simulink model "StampFly_StudentBlocks"  (R2026b)
settings: Solver=VariableStepAuto
undefined symbols (not defined in the file): Bottom, Official
(part 4 of 6)

== system StampFly_StudentBlocks/FlightSequence/OfficialTakeoffHover400/TakeoffHoverControl400/PitchRatePID ==
  Error : Inport
  Dt : Inport  Port=2
  Enable : Inport  Port=3
  Reset : Inport  Port=4
  PreviousError : Inport  Port=5
  ApplyKp : Product
  DMemory : UnitDelay  InitialCondition=single(0)  SampleTime=Official.Step
  DerivativeDenominator : Sum
  DerivativeErrorProduct : Product
  DerivativeErrorTerm : Product  Inputs=*/
  DerivativePreviousNumerator : Sum  Inputs=+-
  DerivativeUpdate : Sum
  DivideTi : Product  Inputs=*/
  EMemory : UnitDelay  InitialCondition=single(0)  SampleTime=Official.Step
  ErrorDifference : Sum  Inputs=+-
  ErrorPair : Sum
  ErrorPairDt : Product
  Eta : Constant  Value=single(0.125)
  EtaTd : Product
  HalfIntegral : Gain  Gain=single(.5)
  IMemory : UnitDelay  InitialCondition=single(0)  SampleTime=Official.Step
  IntegralLimit : Saturate  UpperLimit=single(30000)  LowerLimit=single(-30000)
  IntegralUpdate : Sum
  Kp : Constant  Value=single(0.949999988)
  PIDTerms : Sum  Inputs=+++
  PreviousDerivativeProduct : Product
  PreviousDerivativeTerm : Product  Inputs=*/
  Select_dnext : Switch  Criteria=u2 ~= 0  SaturateOnIntegerOverflow=off  InputSameDT=off
  Select_dp : Switch  Criteria=u2 ~= 0  SaturateOnIntegerOverflow=off  InputSameDT=off
  Select_enext : Switch  Criteria=u2 ~= 0  SaturateOnIntegerOverflow=off  InputSameDT=off
  Select_ep : Switch  Criteria=u2 ~= 0  SaturateOnIntegerOverflow=off  InputSameDT=off
  Select_inext : Switch  Criteria=u2 ~= 0  SaturateOnIntegerOverflow=off  InputSameDT=off
  Select_ip : Switch  Criteria=u2 ~= 0  SaturateOnIntegerOverflow=off  InputSameDT=off
  Select_output : Switch  Criteria=u2 ~= 0  SaturateOnIntegerOverflow=off  InputSameDT=off
  Select_ynext : Switch  Criteria=u2 ~= 0  SaturateOnIntegerOverflow=off  InputSameDT=off
  Td : Constant  Value=single(0.0250000004)
  Ti : Constant  Value=single(0.699999988)
  TwiceEtaTd : Gain  Gain=single(2)
  TwiceTd : Gain  Gain=single(2)
  YMemory : UnitDelay  InitialCondition=single(0)  SampleTime=Official.Step
  Zero : Constant  Value=single(0)
  Output : Outport
  wires:
  Enable/1 -> Select_output/2, Select_inext/2, Select_dnext/2, Select_enext/2, Select_ynext/2
  ApplyKp/1 -> Select_ynext/1, Select_output/1
  YMemory/1 -> Select_ynext/3, Select_output/3
  Select_ynext/1 -> YMemory/1
  Select_output/1 -> Output/1
  Select_enext/1 -> EMemory/1
  Select_dnext/1 -> DMemory/1
  Select_inext/1 -> IMemory/1
  PIDTerms/1 -> ApplyKp/2
  Kp/1 -> ApplyKp/1
  DerivativeUpdate/1 -> PIDTerms/3, Select_dnext/1
  IntegralLimit/1 -> PIDTerms/2, Select_inext/1
  DerivativeErrorTerm/1 -> DerivativeUpdate/2
  PreviousDerivativeTerm/1 -> DerivativeUpdate/1
  DerivativeErrorProduct/1 -> DerivativeErrorTerm/1
  ErrorDifference/1 -> DerivativeErrorProduct/2
  TwiceTd/1 -> DerivativeErrorProduct/1
  DerivativeDenominator/1 -> PreviousDerivativeTerm/2, DerivativeErrorTerm/2
  PreviousDerivativeProduct/1 -> PreviousDerivativeTerm/1
  Select_dp/1 -> PreviousDerivativeProduct/2, Select_dnext/3
  DerivativePreviousNumerator/1 -> PreviousDerivativeProduct/1
  TwiceEtaTd/1 -> DerivativePreviousNumerator/1, DerivativeDenominator/1
  EtaTd/1 -> TwiceEtaTd/1
  Td/1 -> EtaTd/2, TwiceTd/1
  Eta/1 -> EtaTd/1
  IntegralUpdate/1 -> IntegralLimit/1
  DivideTi/1 -> IntegralUpdate/2
  Select_ip/1 -> Select_inext/3, IntegralUpdate/1
  Ti/1 -> DivideTi/2
  HalfIntegral/1 -> DivideTi/1
  ErrorPairDt/1 -> HalfIntegral/1
  ErrorPair/1 -> ErrorPairDt/2
  Dt/1 -> ErrorPairDt/1, DerivativeDenominator/2, DerivativePreviousNumerator/2
  Select_ep/1 -> Select_enext/3, ErrorPair/2, ErrorDifference/2
  Error/1 -> ErrorPair/1, ErrorDifference/1, PIDTerms/1, Select_enext/1
  EMemory/1 -> Select_ep/3
  PreviousError/1 -> Select_ep/1
  DMemory/1 -> Select_dp/3
  IMemory/1 -> Select_ip/3
  Reset/1 -> Select_ip/2, Select_dp/2, Select_ep/2
  Zero/1 -> Select_ip/1, Select_dp/1

== system StampFly_StudentBlocks/FlightSequence/OfficialTakeoffHover400/TakeoffHoverControl400/RollAnglePID ==
  Error : Inport
  Dt : Inport  Port=2
  Enable : Inport  Port=3
  Reset : Inport  Port=4
  PreviousError : Inport  Port=5
  ApplyKp : Product
  DMemory : UnitDelay  InitialCondition=single(0)  SampleTime=Official.Step
  DerivativeDenominator : Sum
  DerivativeErrorProduct : Product
  DerivativeErrorTerm : Product  Inputs=*/
  DerivativePreviousNumerator : Sum  Inputs=+-
  DerivativeUpdate : Sum
  DivideTi : Product  Inputs=*/
  EMemory : UnitDelay  InitialCondition=single(0)  SampleTime=Official.Step
  ErrorDifference : Sum  Inputs=+-
  ErrorPair : Sum
  ErrorPairDt : Product
  Eta : Constant  Value=single(0.125)
  EtaTd : Product
  HalfIntegral : Gain  Gain=single(.5)
  IMemory : UnitDelay  InitialCondition=single(0)  SampleTime=Official.Step
  IntegralLimit : Saturate  UpperLimit=single(30000)  LowerLimit=single(-30000)
  IntegralUpdate : Sum
  Kp : Constant  Value=single(5)
  PIDTerms : Sum  Inputs=+++
  PreviousDerivativeProduct : Product
  PreviousDerivativeTerm : Product  Inputs=*/
  Select_dnext : Switch  Criteria=u2 ~= 0  SaturateOnIntegerOverflow=off  InputSameDT=off
  Select_dp : Switch  Criteria=u2 ~= 0  SaturateOnIntegerOverflow=off  InputSameDT=off
  Select_enext : Switch  Criteria=u2 ~= 0  SaturateOnIntegerOverflow=off  InputSameDT=off
  Select_ep : Switch  Criteria=u2 ~= 0  SaturateOnIntegerOverflow=off  InputSameDT=off
  Select_inext : Switch  Criteria=u2 ~= 0  SaturateOnIntegerOverflow=off  InputSameDT=off
  Select_ip : Switch  Criteria=u2 ~= 0  SaturateOnIntegerOverflow=off  InputSameDT=off
  Select_output : Switch  Criteria=u2 ~= 0  SaturateOnIntegerOverflow=off  InputSameDT=off
  Select_ynext : Switch  Criteria=u2 ~= 0  SaturateOnIntegerOverflow=off  InputSameDT=off
  Td : Constant  Value=single(0.0399999991)
  Ti : Constant  Value=single(4)
  TwiceEtaTd : Gain  Gain=single(2)
  TwiceTd : Gain  Gain=single(2)
  YMemory : UnitDelay  InitialCondition=single(0)  SampleTime=Official.Step
  Zero : Constant  Value=single(0)
  Output : Outport
  wires:
  Enable/1 -> Select_output/2, Select_inext/2, Select_dnext/2, Select_enext/2, Select_ynext/2
  ApplyKp/1 -> Select_ynext/1, Select_output/1
  YMemory/1 -> Select_ynext/3, Select_output/3
  Select_ynext/1 -> YMemory/1
  Select_output/1 -> Output/1
  Select_enext/1 -> EMemory/1
  Select_dnext/1 -> DMemory/1
  Select_inext/1 -> IMemory/1
  PIDTerms/1 -> ApplyKp/2
  Kp/1 -> ApplyKp/1
  DerivativeUpdate/1 -> PIDTerms/3, Select_dnext/1
  IntegralLimit/1 -> PIDTerms/2, Select_inext/1
  DerivativeErrorTerm/1 -> DerivativeUpdate/2
  PreviousDerivativeTerm/1 -> DerivativeUpdate/1
  DerivativeErrorProduct/1 -> DerivativeErrorTerm/1
  ErrorDifference/1 -> DerivativeErrorProduct/2
  TwiceTd/1 -> DerivativeErrorProduct/1
  DerivativeDenominator/1 -> PreviousDerivativeTerm/2, DerivativeErrorTerm/2
  PreviousDerivativeProduct/1 -> PreviousDerivativeTerm/1
  Select_dp/1 -> PreviousDerivativeProduct/2, Select_dnext/3
  DerivativePreviousNumerator/1 -> PreviousDerivativeProduct/1
  TwiceEtaTd/1 -> DerivativePreviousNumerator/1, DerivativeDenominator/1
  EtaTd/1 -> TwiceEtaTd/1
  Td/1 -> EtaTd/2, TwiceTd/1
  Eta/1 -> EtaTd/1
  IntegralUpdate/1 -> IntegralLimit/1
  DivideTi/1 -> IntegralUpdate/2
  Select_ip/1 -> Select_inext/3, IntegralUpdate/1
  Ti/1 -> DivideTi/2
  HalfIntegral/1 -> DivideTi/1
  ErrorPairDt/1 -> HalfIntegral/1
  ErrorPair/1 -> ErrorPairDt/2
  Dt/1 -> ErrorPairDt/1, DerivativeDenominator/2, DerivativePreviousNumerator/2
  Select_ep/1 -> Select_enext/3, ErrorPair/2, ErrorDifference/2
  Error/1 -> ErrorPair/1, ErrorDifference/1, PIDTerms/1, Select_enext/1
  EMemory/1 -> Select_ep/3
  PreviousError/1 -> Select_ep/1
  DMemory/1 -> Select_dp/3
  IMemory/1 -> Select_ip/3
  Reset/1 -> Select_ip/2, Select_dp/2, Select_ep/2
  Zero/1 -> Select_ip/1, Select_dp/1

== system StampFly_StudentBlocks/FlightSequence/OfficialTakeoffHover400/TakeoffHoverControl400/RollRatePID ==
  Error : Inport
  Dt : Inport  Port=2
  Enable : Inport  Port=3
  Reset : Inport  Port=4
  PreviousError : Inport  Port=5
  ApplyKp : Product
  DMemory : UnitDelay  InitialCondition=single(0)  SampleTime=Official.Step
  DerivativeDenominator : Sum
  DerivativeErrorProduct : Product
  DerivativeErrorTerm : Product  Inputs=*/
  DerivativePreviousNumerator : Sum  Inputs=+-
  DerivativeUpdate : Sum
  DivideTi : Product  Inputs=*/
  EMemory : UnitDelay  InitialCondition=single(0)  SampleTime=Official.Step
  ErrorDifference : Sum  Inputs=+-
  ErrorPair : Sum
  ErrorPairDt : Product
  Eta : Constant  Value=single(0.125)
  EtaTd : Product
  HalfIntegral : Gain  Gain=single(.5)
  IMemory : UnitDelay  InitialCondition=single(0)  SampleTime=Official.Step
  IntegralLimit : Saturate  UpperLimit=single(30000)  LowerLimit=single(-30000)
  IntegralUpdate : Sum
  Kp : Constant  Value=single(0.649999976)
  PIDTerms : Sum  Inputs=+++
  PreviousDerivativeProduct : Product
  PreviousDerivativeTerm : Product  Inputs=*/
  Select_dnext : Switch  Criteria=u2 ~= 0  SaturateOnIntegerOverflow=off  InputSameDT=off
  Select_dp : Switch  Criteria=u2 ~= 0  SaturateOnIntegerOverflow=off  InputSameDT=off
  Select_enext : Switch  Criteria=u2 ~= 0  SaturateOnIntegerOverflow=off  InputSameDT=off
  Select_ep : Switch  Criteria=u2 ~= 0  SaturateOnIntegerOverflow=off  InputSameDT=off
  Select_inext : Switch  Criteria=u2 ~= 0  SaturateOnIntegerOverflow=off  InputSameDT=off
  Select_ip : Switch  Criteria=u2 ~= 0  SaturateOnIntegerOverflow=off  InputSameDT=off
  Select_output : Switch  Criteria=u2 ~= 0  SaturateOnIntegerOverflow=off  InputSameDT=off
  Select_ynext : Switch  Criteria=u2 ~= 0  SaturateOnIntegerOverflow=off  InputSameDT=off
  Td : Constant  Value=single(0.00999999978)
  Ti : Constant  Value=single(0.699999988)
  TwiceEtaTd : Gain  Gain=single(2)
  TwiceTd : Gain  Gain=single(2)
  YMemory : UnitDelay  InitialCondition=single(0)  SampleTime=Official.Step
  Zero : Constant  Value=single(0)
  Output : Outport
  wires:
  Enable/1 -> Select_output/2, Select_inext/2, Select_dnext/2, Select_enext/2, Select_ynext/2
  ApplyKp/1 -> Select_ynext/1, Select_output/1
  YMemory/1 -> Select_ynext/3, Select_output/3
  Select_ynext/1 -> YMemory/1
  Select_output/1 -> Output/1
  Select_enext/1 -> EMemory/1
  Select_dnext/1 -> DMemory/1
  Select_inext/1 -> IMemory/1
  PIDTerms/1 -> ApplyKp/2
  Kp/1 -> ApplyKp/1
  DerivativeUpdate/1 -> PIDTerms/3, Select_dnext/1
  IntegralLimit/1 -> PIDTerms/2, Select_inext/1
  DerivativeErrorTerm/1 -> DerivativeUpdate/2
  PreviousDerivativeTerm/1 -> DerivativeUpdate/1
  DerivativeErrorProduct/1 -> DerivativeErrorTerm/1
  ErrorDifference/1 -> DerivativeErrorProduct/2
  TwiceTd/1 -> DerivativeErrorProduct/1
  DerivativeDenominator/1 -> PreviousDerivativeTerm/2, DerivativeErrorTerm/2
  PreviousDerivativeProduct/1 -> PreviousDerivativeTerm/1
  Select_dp/1 -> PreviousDerivativeProduct/2, Select_dnext/3
  DerivativePreviousNumerator/1 -> PreviousDerivativeProduct/1
  TwiceEtaTd/1 -> DerivativePreviousNumerator/1, DerivativeDenominator/1
  EtaTd/1 -> TwiceEtaTd/1
  Td/1 -> EtaTd/2, TwiceTd/1
  Eta/1 -> EtaTd/1
  IntegralUpdate/1 -> IntegralLimit/1
  DivideTi/1 -> IntegralUpdate/2
  Select_ip/1 -> Select_inext/3, IntegralUpdate/1
  Ti/1 -> DivideTi/2
  HalfIntegral/1 -> DivideTi/1
  ErrorPairDt/1 -> HalfIntegral/1
  ErrorPair/1 -> ErrorPairDt/2
  Dt/1 -> ErrorPairDt/1, DerivativeDenominator/2, DerivativePreviousNumerator/2
  Select_ep/1 -> Select_enext/3, ErrorPair/2, ErrorDifference/2
  Error/1 -> ErrorPair/1, ErrorDifference/1, PIDTerms/1, Select_enext/1
  EMemory/1 -> Select_ep/3
  PreviousError/1 -> Select_ep/1
  DMemory/1 -> Select_dp/3
  IMemory/1 -> Select_ip/3
  Reset/1 -> Select_ip/2, Select_dp/2, Select_ep/2
  Zero/1 -> Select_ip/1, Select_dp/1

== system StampFly_StudentBlocks/FlightSequence/OfficialTakeoffHover400/TakeoffHoverControl400/VerticalSpeedPID ==
  Error : Inport
  Dt : Inport  Port=2
  Enable : Inport  Port=3
  Reset : Inport  Port=4
  PreviousError : Inport  Port=5
  ApplyKp : Product
  DMemory : UnitDelay  InitialCondition=single(0)  SampleTime=Official.Step
  DerivativeDenominator : Sum
  DerivativeErrorProduct : Product
  DerivativeErrorTerm : Product  Inputs=*/
  DerivativePreviousNumerator : Sum  Inputs=+-
  DerivativeUpdate : Sum
  DivideTi : Product  Inputs=*/
  EMemory : UnitDelay  InitialCondition=single(0)  SampleTime=Official.Step
  ErrorDifference : Sum  Inputs=+-
  ErrorPair : Sum
  ErrorPairDt : Product
  Eta : Constant  Value=single(0.125)
  EtaTd : Product
  HalfIntegral : Gain  Gain=single(.5)
  IMemory : UnitDelay  InitialCondition=single(0)  SampleTime=Official.Step
  IntegralLimit : Saturate  UpperLimit=single(30000)  LowerLimit=single(-30000)
  IntegralUpdate : Sum
  Kp : Constant  Value=single(0.0799999982)
  PIDTerms : Sum  Inputs=+++
  PreviousDerivativeProduct : Product
  PreviousDerivativeTerm : Product  Inputs=*/
  Select_dnext : Switch  Criteria=u2 ~= 0  SaturateOnIntegerOverflow=off  InputSameDT=off
  Select_dp : Switch  Criteria=u2 ~= 0  SaturateOnIntegerOverflow=off  InputSameDT=off
  Select_enext : Switch  Criteria=u2 ~= 0  SaturateOnIntegerOverflow=off  InputSameDT=off
  Select_ep : Switch  Criteria=u2 ~= 0  SaturateOnIntegerOverflow=off  InputSameDT=off
  Select_inext : Switch  Criteria=u2 ~= 0  SaturateOnIntegerOverflow=off  InputSameDT=off
  Select_ip : Switch  Criteria=u2 ~= 0  SaturateOnIntegerOverflow=off  InputSameDT=off
  Select_output : Switch  Criteria=u2 ~= 0  SaturateOnIntegerOverflow=off  InputSameDT=off
  Select_ynext : Switch  Criteria=u2 ~= 0  SaturateOnIntegerOverflow=off  InputSameDT=off
  Td : Constant  Value=single(0.0799999982)
  Ti : Constant  Value=single(0.949999988)
  TwiceEtaTd : Gain  Gain=single(2)
  TwiceTd : Gain  Gain=single(2)
  YMemory : UnitDelay  InitialCondition=single(0)  SampleTime=Official.Step
  Zero : Constant  Value=single(0)
  Output : Outport
  wires:
  Enable/1 -> Select_output/2, Select_inext/2, Select_dnext/2, Select_enext/2, Select_ynext/2
  ApplyKp/1 -> Select_ynext/1, Select_output/1
  YMemory/1 -> Select_ynext/3, Select_output/3
  Select_ynext/1 -> YMemory/1
  Select_output/1 -> Output/1
  Select_enext/1 -> EMemory/1
  Select_dnext/1 -> DMemory/1
  Select_inext/1 -> IMemory/1
  PIDTerms/1 -> ApplyKp/2
  Kp/1 -> ApplyKp/1
  DerivativeUpdate/1 -> PIDTerms/3, Select_dnext/1
  IntegralLimit/1 -> PIDTerms/2, Select_inext/1
  DerivativeErrorTerm/1 -> DerivativeUpdate/2
  PreviousDerivativeTerm/1 -> DerivativeUpdate/1
  DerivativeErrorProduct/1 -> DerivativeErrorTerm/1
  ErrorDifference/1 -> DerivativeErrorProduct/2
  TwiceTd/1 -> DerivativeErrorProduct/1
  DerivativeDenominator/1 -> PreviousDerivativeTerm/2, DerivativeErrorTerm/2
  PreviousDerivativeProduct/1 -> PreviousDerivativeTerm/1
  Select_dp/1 -> PreviousDerivativeProduct/2, Select_dnext/3
  DerivativePreviousNumerator/1 -> PreviousDerivativeProduct/1
  TwiceEtaTd/1 -> DerivativePreviousNumerator/1, DerivativeDenominator/1
  EtaTd/1 -> TwiceEtaTd/1
  Td/1 -> EtaTd/2, TwiceTd/1
  Eta/1 -> EtaTd/1
  IntegralUpdate/1 -> IntegralLimit/1
  DivideTi/1 -> IntegralUpdate/2
  Select_ip/1 -> Select_inext/3, IntegralUpdate/1
  Ti/1 -> DivideTi/2
  HalfIntegral/1 -> DivideTi/1
  ErrorPairDt/1 -> HalfIntegral/1
  ErrorPair/1 -> ErrorPairDt/2
  Dt/1 -> ErrorPairDt/1, DerivativeDenominator/2, DerivativePreviousNumerator/2
  Select_ep/1 -> Select_enext/3, ErrorPair/2, ErrorDifference/2
  Error/1 -> ErrorPair/1, ErrorDifference/1, PIDTerms/1, Select_enext/1
  EMemory/1 -> Select_ep/3
  PreviousError/1 -> Select_ep/1
  DMemory/1 -> Select_dp/3
  IMemory/1 -> Select_ip/3
  Reset/1 -> Select_ip/2, Select_dp/2, Select_ep/2
  Zero/1 -> Select_ip/1, Select_dp/1

== system StampFly_StudentBlocks/FlightSequence/OfficialTakeoffHover400/TakeoffHoverControl400/YawRatePID ==
  Error : Inport
  Dt : Inport  Port=2
  Enable : Inport  Port=3
  Reset : Inport  Port=4
  PreviousError : Inport  Port=5
  ApplyKp : Product
  DMemory : UnitDelay  InitialCondition=single(0)  SampleTime=Official.Step
  DerivativeDenominator : Sum
  DerivativeErrorProduct : Product
  DerivativeErrorTerm : Product  Inputs=*/
  DerivativePreviousNumerator : Sum  Inputs=+-
  DerivativeUpdate : Sum
  DivideTi : Product  Inputs=*/
  EMemory : UnitDelay  InitialCondition=single(0)  SampleTime=Official.Step
  ErrorDifference : Sum  Inputs=+-
  ErrorPair : Sum
  ErrorPairDt : Product
  Eta : Constant  Value=single(0.125)
  EtaTd : Product
  HalfIntegral : Gain  Gain=single(.5)
  IMemory : UnitDelay  InitialCondition=single(0)  SampleTime=Official.Step
  IntegralLimit : Saturate  UpperLimit=single(30000)  LowerLimit=single(-30000)
  IntegralUpdate : Sum
  Kp : Constant  Value=single(3)
  PIDTerms : Sum  Inputs=+++
  PreviousDerivativeProduct : Product
  PreviousDerivativeTerm : Product  Inputs=*/
  Select_dnext : Switch  Criteria=u2 ~= 0  SaturateOnIntegerOverflow=off  InputSameDT=off
  Select_dp : Switch  Criteria=u2 ~= 0  SaturateOnIntegerOverflow=off  InputSameDT=off
  Select_enext : Switch  Criteria=u2 ~= 0  SaturateOnIntegerOverflow=off  InputSameDT=off
  Select_ep : Switch  Criteria=u2 ~= 0  SaturateOnIntegerOverflow=off  InputSameDT=off
  Select_inext : Switch  Criteria=u2 ~= 0  SaturateOnIntegerOverflow=off  InputSameDT=off
  Select_ip : Switch  Criteria=u2 ~= 0  SaturateOnIntegerOverflow=off  InputSameDT=off
  Select_output : Switch  Criteria=u2 ~= 0  SaturateOnIntegerOverflow=off  InputSameDT=off
  Select_ynext : Switch  Criteria=u2 ~= 0  SaturateOnIntegerOverflow=off  InputSameDT=off
  Td : Constant  Value=single(0.00999999978)
  Ti : Constant  Value=single(0.800000012)
  TwiceEtaTd : Gain  Gain=single(2)
  TwiceTd : Gain  Gain=single(2)
  YMemory : UnitDelay  InitialCondition=single(0)  SampleTime=Official.Step
  Zero : Constant  Value=single(0)
  Output : Outport
  wires:
  Enable/1 -> Select_output/2, Select_inext/2, Select_dnext/2, Select_enext/2, Select_ynext/2
  ApplyKp/1 -> Select_ynext/1, Select_output/1
  YMemory/1 -> Select_ynext/3, Select_output/3
  Select_ynext/1 -> YMemory/1
  Select_output/1 -> Output/1
  Select_enext/1 -> EMemory/1
  Select_dnext/1 -> DMemory/1
  Select_inext/1 -> IMemory/1
  PIDTerms/1 -> ApplyKp/2
  Kp/1 -> ApplyKp/1
  DerivativeUpdate/1 -> PIDTerms/3, Select_dnext/1
  IntegralLimit/1 -> PIDTerms/2, Select_inext/1
  DerivativeErrorTerm/1 -> DerivativeUpdate/2
  PreviousDerivativeTerm/1 -> DerivativeUpdate/1
  DerivativeErrorProduct/1 -> DerivativeErrorTerm/1
  ErrorDifference/1 -> DerivativeErrorProduct/2
  TwiceTd/1 -> DerivativeErrorProduct/1
  DerivativeDenominator/1 -> PreviousDerivativeTerm/2, DerivativeErrorTerm/2
  PreviousDerivativeProduct/1 -> PreviousDerivativeTerm/1
  Select_dp/1 -> PreviousDerivativeProduct/2, Select_dnext/3
  DerivativePreviousNumerator/1 -> PreviousDerivativeProduct/1
  TwiceEtaTd/1 -> DerivativePreviousNumerator/1, DerivativeDenominator/1
  EtaTd/1 -> TwiceEtaTd/1
  Td/1 -> EtaTd/2, TwiceTd/1
  Eta/1 -> EtaTd/1
  IntegralUpdate/1 -> IntegralLimit/1
  DivideTi/1 -> IntegralUpdate/2
  Select_ip/1 -> Select_inext/3, IntegralUpdate/1
  Ti/1 -> DivideTi/2
  HalfIntegral/1 -> DivideTi/1
  ErrorPairDt/1 -> HalfIntegral/1
  ErrorPair/1 -> ErrorPairDt/2
  Dt/1 -> ErrorPairDt/1, DerivativeDenominator/2, DerivativePreviousNumerator/2
  Select_ep/1 -> Select_enext/3, ErrorPair/2, ErrorDifference/2
  Error/1 -> ErrorPair/1, ErrorDifference/1, PIDTerms/1, Select_enext/1
  EMemory/1 -> Select_ep/3
  PreviousError/1 -> Select_ep/1
  DMemory/1 -> Select_dp/3
  IMemory/1 -> Select_ip/3
  Reset/1 -> Select_ip/2, Select_dp/2, Select_ep/2
  Zero/1 -> Select_ip/1, Select_dp/1

== stateflow chart StampFly_StudentBlocks/Estimation/MadgwickAttitude ==
  note: Madgwick姿勢推定：400 Hz、β=0.1。公式の高速逆平方根、軸の対応、Yaw+180°を保持。数式はこのChart内にあります。
  state Calculate
    en: [a,q]=stepFn(rates,accel,mode,reset);
    du: [a,q]=stepFn(rates,accel,mode,reset);
  (default) -> Calculate
  data: arg_rates function_input; arg_accel function_input; arg_mode function_input; arg_reset function_input; arg_a function_output; arg_q function_output; rates input single; accel input single; mode input uint8; reset input boolean; a output single; q output single
  function [arg_a,arg_q]=stepFn(arg_rates,arg_accel,arg_mode,arg_reset):
    | function [arg_a,arg_q]=stepFn(arg_rates,arg_accel,arg_mode,arg_reset)
    | % 日本語の説明はブロック注釈とDescriptionを参照。
    | %#codegen
    | persistent Q Angles;
    | if isempty(Q)
    | Q=single([1;0;0;0]);
    | Angles=zeros(3,1,'single');
    | end
    |             if arg_reset,Q=single([1;0;0;0]);end
    |             if arg_mode>1,[Angles,Q]=madgwickStep(arg_rates,arg_accel,Q,false);end
    |             arg_a=Angles;arg_q=Q;
    | end
    | 
    | function [attitude,arg_q] = madgwickStep(arg_rates,arg_accel,arg_q,arg_reset)
    | %MADGWICKSTEP Official updateIMU with body-axis conventions and invSqrt.
    | % Rates rad/s and arg_accel g in official body frame [forward;left;down].
    | % Madgwick is fixed 400 Hz even though other official filters use measured dt.
    | % Translation of lib/MdgwickAHRS/MadgwickAHRS.cpp; original license retained.
    | %#codegen
    | if arg_reset, arg_q=single([1;0;0;0]); end
    | q0=arg_q(1);q1=arg_q(2);q2=arg_q(3);q3=arg_q(4);
    | % Retain original rad->deg->rad conversion coefficients, including rounding.
    | g=arg_rates([2 1 3])*single(180/pi);g(3)=-g(3);
    | g=g*single(0.0174533);gx=g(1);gy=g(2);gz=g(3);
    | arg_a=arg_accel([2 1 3]);arg_a(3)=-arg_a(3);ax=arg_a(1);ay=arg_a(2);az=arg_a(3);
    | dq=single(0.5)*[-q1*gx-q2*gy-q3*gz; q0*gx+q2*gz-q3*gy; ...
    |     q0*gy-q1*gz+q3*gx; q0*gz+q1*gy-q2*gx];
    | if ax~=0 || ay~=0 || az~=0
    |     reciprocal=fastInvSqrt(ax*ax+ay*ay+az*az);
    |     ax=ax*reciprocal;ay=ay*reciprocal;az=az*reciprocal;
    |     q02=q0*q0;q12=q1*q1;q22=q2*q2;q32=q3*q3;
    |     q0x2=single(2)*q0;q1x2=single(2)*q1;q2x2=single(2)*q2;q3x2=single(2)*q3;
    |     q0x4=single(4)*q0;q1x4=single(4)*q1;q2x4=single(4)*q2;
    |     q1x8=single(8)*q1;q2x8=single(8)*q2;
    |     gradient=[q0x4*q22+q2x2*ax+q0x4*q12-q1x2*ay; ...
    |         q1x4*q32-q3x2*ax+single(4)*q02*q1-q0x2*ay-q1x4+q1x8*q12+q1x8*q22+q1x4*az; ...
    |         single(4)*q02*q2+q0x2*ax+q2x4*q32-q3x2*ay-q2x4+q2x8*q12+q2x8*q22+q2x4*az; ...
    |         single(4)*q12*q3-q1x2*ax+single(4)*q22*q3-q2x2*ay];
    |     reciprocal=fastInvSqrt(gradient(1)*gradient(1)+gradient(2)*gradient(2)+gradient(3)*gradient(3)+gradient(4)*gradient(4));
    |     gradient=gradient*reciprocal;
    |     dq=dq-single(0.1)*gradient;
    | end
    | arg_q=arg_q+dq*single(1/400);
    | reciprocal=fastInvSqrt(arg_q(1)*arg_q(1)+arg_q(2)*arg_q(2)+arg_q(3)*arg_q(3)+arg_q(4)*arg_q(4));arg_q=arg_q*reciprocal;
    | roll=atan2(arg_q(1)*arg_q(2)+arg_q(3)*arg_q(4),single(0.5)-arg_q(2)*arg_q(2)-arg_q(3)*arg_q(3));
    | pitch=asin(-single(2)*(arg_q(2)*arg_q(4)-arg_q(1)*arg_q(3)));
    | yaw=atan2(arg_q(2)*arg_q(3)+arg_q(1)*arg_q(4),single(0.5)-arg_q(3)*arg_q(3)-arg_q(4)*arg_q(4));
    | % Original getYaw adds 180 degrees; do not hide this offset.
    | attitude=[pitch*single(57.29578);roll*single(57.29578); ...
    |     -(yaw*single(57.29578)+single(180))]*single(pi/180);
    | end
    | 
    | function y=fastInvSqrt(x)
    | i=typecast(x,'uint32');i=uint32(hex2dec('5f3759df'))-bitshift(i,-1);
    | y=typecast(i,'single');half=single(0.5)*x;
    | y=y*(single(1.5)-half*y*y);y=y*(single(1.5)-half*y*y);
    | end

== stateflow chart StampFly_StudentBlocks/Controllers/TakeoffHoverControl400/ControlDiagnosticPack ==
  state Calculate
    en: [diag]=stepFn(alt,base,counter,zRef,thrust,angle,rate,rollTorque,pitchTorque,yawTorque,before);
    du: [diag]=stepFn(alt,base,counter,zRef,thrust,angle,rate,rollTorque,pitchTorque,yawTorque,before);
  (default) -> Calculate
  data: alt function_input; base function_input; counter function_input; zRef function_input; thrust function_input; angle function_input; rate function_input; rollTorque function_input; pitchTorque function_input; yawTorque function_input; before function_input; diag function_output; alt input single; base input single; counter input uint16; zRef input single; thrust input single; angle input single; rate input single; rollTorque input single; pitchTorque input single; yawTorque input single; before input single; diag output single
  function diag =stepFn(alt,base,counter,zRef,thrust,angle,rate,rollTorque,pitchTorque,yawTorque,before):
    | function diag =stepFn(alt,base,counter,zRef,thrust,angle,rate,rollTorque,pitchTorque,yawTorque,before)
    | % 日本語の説明はブロック注釈とDescriptionを参照。
    | %#codegen
    |             diag=[alt;base;single(counter);zRef;thrust;angle;rate;rollTorque;pitchTorque;yawTorque;before];
    | end

== stateflow chart StampFly_StudentBlocks/Controllers/TakeoffHoverControl400/ControlEnableReset ==
  note: 実行/リセット判定：推力Dutyが0.1未満ならPIDをリセットし、各ループのEnableを決めます。
  state Calculate
    en: [command,run,reset,altEnable,angleEnable,velEnable,angleReset,flipFlag]=stepFn(raw,manual,auto,mode,controlMode,dt,oldFilter,lastThrust,phase,flipThrust,flipStart,flipDone,finalMode);
    du: [command,run,reset,altEnable,angleEnable,velEnable,angleReset,flipFlag]=stepFn(raw,manual,auto,mode,controlMode,dt,oldFilter,lastThrust,phase,flipThrust,flipStart,flipDone,finalMode);
  (default) -> Calculate
  data: arg_arg_raw function_input; arg_arg_manual function_input; arg_arg_auto function_input; arg_branch function_input; arg_arg_controlMode function_input; arg_arg_dt function_input; arg_arg_oldFilter function_input; arg_arg_lastThrust function_input; arg_arg_command function_output; arg_arg_run function_output; arg_arg_reset function_output; arg_arg_altEnable function_output; arg_arg_angleEnable function_output; arg_arg_velEnable function_output; arg_arg_phase function_input; arg_arg_flipThrust function_input; arg_arg_flipStart function_input; arg_arg_flipDone function_input; arg_arg_mode function_input; arg_arg_angleReset function_output; arg_arg_flipFlag function_output; raw input single; manual input boolean; auto input boolean; mode input uint8; controlMode input single; dt input single; oldFilter input single; lastThrust input single; command output single; run output boolean; reset output boolean; altEnable output boolean; angleEnable output boolean; velEnable output boolean; phase input uint8; flipThrust input single; flipStart input boolean; flipDone input boolean; finalMode input uint8; angleReset output boolean; flipFlag output uint8
  function [arg_arg_command,arg_arg_run,arg_arg_reset,arg_arg_altEnable,arg_arg_angleEnable,arg_arg_velEnable,arg_arg_angleReset,arg_arg_flipFlag]=stepFn(arg_arg_raw,arg_arg_manual,arg_arg_auto,arg_branch,arg_arg_controlMode,arg_arg_dt,arg_arg_oldFilter,arg_arg_lastThrust,arg_arg_phase,arg_arg_flipThrust,arg_arg_flipStart,arg_arg_flipDone,arg_arg_mode):
    | function [arg_arg_command,arg_arg_run,arg_arg_reset,arg_arg_altEnable,arg_arg_angleEnable,arg_arg_velEnable,arg_arg_angleReset,arg_arg_flipFlag]=stepFn(arg_arg_raw,arg_arg_manual,arg_arg_auto,arg_branch,arg_arg_controlMode,arg_arg_dt,arg_arg_oldFilter,arg_arg_lastThrust,arg_arg_phase,arg_arg_flipThrust,arg_arg_flipStart,arg_arg_flipDone,arg_arg_mode)
    | % angle_controlとrate_controlで異なるリセット条件を保持する。
    | %#codegen
    | persistent heldFlip;
    | if isempty(heldFlip),heldFlip=uint8(0);end
    | arg_arg_command=arg_arg_raw;
    | if arg_arg_manual,arg_arg_command=filterStep(arg_arg_raw,arg_arg_dt,single(.01),arg_arg_oldFilter);end
    | if arg_branch==5 || arg_branch==3 || arg_arg_flipDone,arg_arg_command=arg_arg_lastThrust;end
    | if arg_branch==6 && arg_arg_phase>0,arg_arg_command=arg_arg_flipThrust;end
    | active=arg_branch==2 || arg_branch==5 || (arg_branch==6 && ~arg_arg_flipDone);
    | angleCalled=active && (arg_arg_phase==0 || arg_arg_phase==1);
    | arg_arg_angleReset=angleCalled && double(arg_arg_command)/3.7<double(single(.1));
    | arg_arg_flipFlag=heldFlip;
    | if arg_branch==3 || arg_arg_flipDone,arg_arg_flipFlag=uint8(0);end
    | if arg_branch==6 && ~arg_arg_flipDone,arg_arg_flipFlag=arg_arg_phase;end
    | if arg_arg_flipStart,arg_arg_flipFlag=uint8(1);end
    | if arg_arg_angleReset,arg_arg_flipFlag=uint8(0);end
    | arg_arg_reset=active && double(arg_arg_command)/3.7<double(single(.1)) && arg_arg_flipFlag==0;
    | arg_arg_run=active && ~arg_arg_reset;
    | arg_arg_altEnable=angleCalled && ~arg_arg_angleReset && arg_arg_auto;
    | arg_arg_angleEnable=angleCalled && ~arg_arg_angleReset && uint8(arg_arg_controlMode)==0;
    | arg_arg_velEnable=arg_arg_run && ((arg_arg_auto && arg_arg_flipFlag==0) || arg_arg_mode==5);
    | if arg_arg_reset,arg_arg_flipFlag=uint8(0);end
    | heldFlip=arg_arg_flipFlag;
    | end
    | function s=filterStep(u,h,T,s),s=s*T/(T+h)+u*h/(T+h);end

== stateflow chart StampFly_StudentBlocks/Controllers/TakeoffHoverControl400/FinalizeFlightMode ==
  state Calculate
    en: [mode]=stepFn(branch,preMode,height,flipStart,flipDone,overG);
    du: [mode]=stepFn(branch,preMode,height,flipStart,flipDone,overG);
  (default) -> Calculate
  data: arg_branch function_input; arg_preMode function_input; arg_height function_input; arg_flipStart function_input; arg_flipDone function_input; arg_overG function_input; arg_mode function_output; branch input uint8; preMode input uint8; height input single; flipStart input boolean; flipDone input boolean; overG input uint8; mode output uint8
  function arg_mode=stepFn(arg_branch,arg_preMode,arg_height,arg_flipStart,arg_flipDone,arg_overG):
    | function arg_mode=stepFn(arg_branch,arg_preMode,arg_height,arg_flipStart,arg_flipDone,arg_overG)
    | % loop分岐の途中で変わるMode。get_commandは分岐途中でもFlipに変更できる。
    | %#codegen
    | arg_mode=arg_preMode;
    | if arg_branch==5 && arg_height<.1,arg_mode=uint8(3);end
    | if arg_flipStart && (arg_branch==2 || arg_branch==6),arg_mode=uint8(6);end
    | if arg_branch==6 && arg_flipDone,arg_mode=uint8(2);end
    | if (arg_branch==2 || arg_branch==5 || arg_branch==6) && arg_overG==1,arg_mode=uint8(3);end
    | end

== stateflow chart StampFly_StudentBlocks/Controllers/TakeoffHoverControl400/SelectRateReference ==
  state Calculate
    en: [rate]=stepFn(direct,rollPID,pitchPID,angleEnable);
    du: [rate]=stepFn(direct,rollPID,pitchPID,angleEnable);
  (default) -> Calculate
  data: direct function_input; rollPID function_input; pitchPID function_input; angleEnable function_input; rate function_output; direct input single; rollPID input single; pitchPID input single; angleEnable input boolean; rate output single
  function rate =stepFn(direct,rollPID,pitchPID,angleEnable):
    | function rate =stepFn(direct,rollPID,pitchPID,angleEnable)
    | % 日本語の説明はブロック注釈とDescriptionを参照。
    | %#codegen
    |             rate=direct;if angleEnable,rate(1)=rollPID;rate(2)=pitchPID;end
    | end

== stateflow chart StampFly_StudentBlocks/Controllers/TakeoffHoverControl400/SelectVerticalReference ==
  state Calculate
    en: [vRef]=stepFn(zRef,mode,auto,flipFlag);
    du: [vRef]=stepFn(zRef,mode,auto,flipFlag);
  (default) -> Calculate
  data: arg_zRef function_input; arg_mode function_input; arg_vRef function_output; arg_auto function_input; arg_flipFlag function_input; zRef input single; mode input uint8; vRef output single; auto input boolean; flipFlag input uint8
  function arg_vRef=stepFn(arg_zRef,arg_mode,arg_auto,arg_flipFlag):
    | function arg_vRef=stepFn(arg_zRef,arg_mode,arg_auto,arg_flipFlag)
    | % Auto高度補正が優先。公式else-ifの順序を維持。
    | %#codegen
    | arg_vRef=arg_zRef;if ~(arg_auto && arg_flipFlag==0) && arg_mode==5,arg_vRef=single(-.15);end
    | end

== stateflow chart StampFly_StudentBlocks/Controllers/TakeoffHoverControl400/StickToAngleRate ==
  note: スティック→目標：Stabilizeは角度±30°、Sportは角速度カーブ。中立位置は低推力時に保存。Yawは角速度指令。
  state Calculate
    en: [angle,directRate,resetError]=stepFn(stick,mode,run,reset,phase,flipRate,angleReset,lastRate,flipDone,controlMode);
    du: [angle,directRate,resetError]=stepFn(stick,mode,run,reset,phase,flipRate,angleReset,lastRate,flipDone,controlMode);
  (default) -> Calculate
  data: arg_arg_stick function_input; arg_branch function_input; arg_arg_run function_input; arg_arg_reset function_input; arg_arg_angle function_output; arg_arg_directRate function_output; arg_arg_resetError function_output; arg_arg_phase function_input; arg_arg_flipRate function_input; arg_arg_angleReset function_input; arg_arg_lastRate function_input; arg_arg_flipDone function_input; arg_arg_controlMode function_input; stick input single; mode input uint8; run input boolean; reset input boolean; angle output single; directRate output single; resetError output single; phase input uint8; flipRate input single; angleReset input boolean; lastRate input single; flipDone input boolean; controlMode input single
  function [arg_arg_angle,arg_arg_directRate,arg_arg_resetError]=stepFn(arg_arg_stick,arg_branch,arg_arg_run,arg_arg_reset,arg_arg_phase,arg_arg_flipRate,arg_arg_angleReset,arg_arg_lastRate,arg_arg_flipDone,arg_arg_controlMode):
    | function [arg_arg_angle,arg_arg_directRate,arg_arg_resetError]=stepFn(arg_arg_stick,arg_branch,arg_arg_run,arg_arg_reset,arg_arg_phase,arg_arg_flipRate,arg_arg_angleReset,arg_arg_lastRate,arg_arg_flipDone,arg_arg_controlMode)
    | % command、角度目標、中立点を別々に保持。Sportは角度commandを更新しない。
    | %#codegen
    | persistent Angle Centers AngleCmd YawCmd;
    | if isempty(Angle),Angle=zeros(2,1,'single');Centers=zeros(3,1,'single');AngleCmd=zeros(2,1,'single');YawCmd=single(0);end
    | arg_arg_directRate=arg_arg_lastRate;arg_arg_resetError=Angle;
    | commandCalled=arg_branch==2 || arg_branch==5 || (arg_branch==6 && arg_arg_phase==0 && ~arg_arg_flipDone);
    | if commandCalled
    |  if uint8(arg_arg_controlMode)==0 || arg_branch==5,AngleCmd=min(max(single(.4*double(arg_arg_stick(1:2))),single(-1)),single(1));end
    |  YawCmd=min(max(arg_arg_stick(3),single(-1)),single(1));
    |  arg_arg_directRate(3)=single(2*pi*double(YawCmd-Centers(3)));
    |  if uint8(arg_arg_controlMode)==1,arg_arg_directRate(1)=rateCommand(arg_arg_stick(1));arg_arg_directRate(2)=rateCommand(arg_arg_stick(2));end
    | elseif arg_branch==6 && arg_arg_phase==1,AngleCmd(:)=single(0);
    | end
    | if arg_arg_angleReset,Centers(1:2)=AngleCmd;end
    | if arg_arg_reset,Centers(3)=YawCmd;end
    | if arg_arg_run && (arg_arg_phase==0 || arg_arg_phase==1) && uint8(arg_arg_controlMode)==0
    |  limit=single(30*pi/180);Angle=min(max(single(.5*pi*double(AngleCmd-Centers(1:2))),-limit),limit);
    | end
    | if arg_branch==6 && arg_arg_phase>=2,arg_arg_directRate(1)=arg_arg_flipRate;arg_arg_directRate(2)=single(0);end
    | if arg_branch==3,arg_arg_directRate(1)=single(0);end
    | if arg_arg_reset,arg_arg_directRate(:)=single(0);end
    | arg_arg_angle=Angle;
    | end
    | function y=rateCommand(x)
    | x=min(max(x,single(-1)),single(1));a=abs(x);t=a*(a*a*a*a*a*single(.5)+a*single(.5));
    | y=single(pi/180)*((single(1600)-single(70))*t+single(70)*a);if x<0,y=-y;end
    | end

== stateflow chart StampFly_StudentBlocks/Estimation/VerticalAcceleration ==
  note: 鉛直加速度：校正後AccelZ差分を反転して100 msフィルター。公式に合わせ単位gのまま高度Kalmanへ入力。
  state Calculate
    en: [az]=stepFn(azd,mode,dt);
    du: [az]=stepFn(azd,mode,dt);
  (default) -> Calculate
  data: azd function_input; mode function_input; dt function_input; az function_output; azd input single; mode input uint8; dt input single; az output single
  function az =stepFn(azd,mode,dt):
    | function az =stepFn(azd,mode,dt)
    | % 日本語の説明はブロック注釈とDescriptionを参照。
    | %#codegen
    | persistent Az PreviousMode;
    | if isempty(Az)
    | Az=single(0);
    | PreviousMode=uint8(0);
    | end
    |             if mode==3 && mode~=PreviousMode,Az=single(0);end
    |             if mode>1,Az=filterStep(-azd,dt,single(0.1),Az);end
    |             az=Az;PreviousMode=mode;
    | end
    | 
    | function s = filterStep(u,h,T,s)
    | %FILTERSTEP Exact Filter::update, including operation ordering.
    | %#codegen
    | s = s*T/(T+h) + u*h/(T+h);
    | end

== stateflow chart StampFly_StudentBlocks/Controllers/TakeoffHoverControl400/TakeoffLandingCommand ==
  note: 離陸/着陸の指令：離陸カウンター0〜1000、初期高度0.5 m、上下スティックで0.05〜1.8 m。電圧トリム=-0.2448V+1.5892。
  state Calculate
    en: [alt,base,counter,raw,auto,manual,controlMode]=stepFn(stick,height,voltage,rangeFlag,mode,phase,flipDone);
    du: [alt,base,counter,raw,auto,manual,controlMode]=stepFn(stick,height,voltage,rangeFlag,mode,phase,flipDone);
  (default) -> Calculate
  data: arg_arg_stick function_input; arg_arg_height function_input; arg_arg_voltage function_input; arg_arg_rangeFlag function_input; arg_branch function_input; arg_arg_alt function_output; arg_arg_base function_output; arg_arg_counter function_output; arg_arg_raw function_output; arg_arg_auto function_output; arg_arg_manual function_output; arg_arg_phase function_input; arg_arg_flipDone function_input; arg_arg_controlMode function_output; stick input single; height input single; voltage input single; rangeFlag input uint8; mode input uint8; alt output single; base output single; counter output uint16; raw output single; auto output boolean; manual output boolean; phase input uint8; flipDone input boolean; controlMode output single
  function [arg_arg_alt,arg_arg_base,arg_arg_counter,arg_arg_raw,arg_arg_auto,arg_arg_manual,arg_arg_controlMode]=stepFn(arg_arg_stick,arg_arg_height,arg_arg_voltage,arg_arg_rangeFlag,arg_branch,arg_arg_phase,arg_arg_flipDone):
    | function [arg_arg_alt,arg_arg_base,arg_arg_counter,arg_arg_raw,arg_arg_auto,arg_arg_manual,arg_arg_controlMode]=stepFn(arg_arg_stick,arg_arg_height,arg_arg_voltage,arg_arg_rangeFlag,arg_branch,arg_arg_phase,arg_arg_flipDone)
    | % 公式get_command/auto_landing。Alt_flagはManual切替時にも保持される。
    | %#codegen
    | persistent Alt Base Counter RangeOld Landing History AltFlag ControlMode;
    | if isempty(Alt)
    |  Alt=single(.5);Base=single(0);Counter=uint16(0);RangeOld=uint8(0);
    |  Landing=false;History=zeros(10,1,'single');AltFlag=false;ControlMode=uint8(0);
    | end
    | arg_arg_raw=single(0);arg_arg_manual=false;
    | if arg_branch==3
    |  Base=single(0);Alt=single(.5);Counter=uint16(0);Landing=false;AltFlag=false;
    | elseif arg_branch==2 || (arg_branch==6 && arg_arg_phase==0 && ~arg_arg_flipDone)
    |  ControlMode=uint8(arg_arg_stick(5));
    |  if uint8(arg_arg_stick(6))==4
    |   AltFlag=true;
    |   if Counter<500
    |    Base=min(single(Counter)/single(1000),trim(single(3.8)));Counter=Counter+uint16(1);
    |   elseif Counter<1000
    |    Base=min(single(Counter)/single(1000),trim(arg_arg_voltage));Counter=Counter+uint16(1);
    |   else,Base=trim(arg_arg_voltage);end
    |   th=arg_arg_stick(4);if th>-.2 && th<.2,th=single(0);end
    |   Alt=min(max(single(double(Alt)+double(th)*.001),single(.05)),single(1.8));
    |   if arg_arg_rangeFlag>RangeOld || arg_arg_rangeFlag==20,Base=Base-single(.02);RangeOld=arg_arg_rangeFlag;end
    |   arg_arg_raw=single(double(Base)*3.7);
    |  else
    |   arg_arg_manual=true;th=min(max(arg_arg_stick(4),single(0)),single(1));
    |   if th>-.2 && th<.2,th=single(0);end
    |   arg_arg_raw=single((.00413+double(single(3.3)*th-single(5.44)*th*th+single(3.13)*th*th*th))*3.7);
    |  end
    | elseif arg_branch==5
    |  AltFlag=false;
    |  if ~Landing,Landing=true;History(:)=arg_arg_height;Base=trim(arg_arg_voltage);end
    |  if History(10)>=arg_arg_height,Base=single(double(Base)*.9999);end
    |  if arg_arg_height<.15,Base=single(double(Base)*.999);end
    |  if arg_arg_height<.1,Landing=false;end
    |  for j=2:10,History(j)=History(j-1);end
    |  History(1)=arg_arg_height;
    | end
    | arg_arg_alt=Alt;arg_arg_base=Base;arg_arg_counter=Counter;arg_arg_auto=AltFlag;arg_arg_controlMode=single(ControlMode);
    | end
    | function y=trim(v),y=-single(.2448)*v+single(1.5892);end

== stateflow chart StampFly_StudentBlocks/Controllers/TakeoffHoverControl400/ThrustCorrectionLimits ==
  note: 鉛直速度PID補正から推力を生成。10 msフィルター後、Auto高度では基準推力の0.85〜1.15倍に制限。
  state Calculate
    en: [thrust,filter,last]=stepFn(command,correction,base,auto,manual,velEnable,mode,dt,oldFilter,lastThrust,flipFlag);
    du: [thrust,filter,last]=stepFn(command,correction,base,auto,manual,velEnable,mode,dt,oldFilter,lastThrust,flipFlag);
  (default) -> Calculate
  data: arg_arg_command function_input; arg_arg_correction function_input; arg_arg_base function_input; arg_arg_auto function_input; arg_arg_manual function_input; arg_arg_velEnable function_input; arg_branch function_input; arg_arg_dt function_input; arg_arg_oldFilter function_input; arg_arg_lastThrust function_input; arg_arg_thrust function_output; arg_arg_filter function_output; arg_arg_last function_output; arg_arg_flipFlag function_input; command input single; correction input single; base input single; auto input boolean; manual input boolean; velEnable input boolean; mode input uint8; dt input single; oldFilter input single; lastThrust input single; thrust output single; filter output single; last output single; flipFlag input uint8
  function [arg_arg_thrust,arg_arg_filter,arg_arg_last]=stepFn(arg_arg_command,arg_arg_correction,arg_arg_base,arg_arg_auto,arg_arg_manual,arg_arg_velEnable,arg_branch,arg_arg_dt,arg_arg_oldFilter,arg_arg_lastThrust,arg_arg_flipFlag):
    | function [arg_arg_thrust,arg_arg_filter,arg_arg_last]=stepFn(arg_arg_command,arg_arg_correction,arg_arg_base,arg_arg_auto,arg_arg_manual,arg_arg_velEnable,arg_branch,arg_arg_dt,arg_arg_oldFilter,arg_arg_lastThrust,arg_arg_flipFlag)
    | % rate_control: Auto補正がLanding補正より優先。Flip中はAuto補正を停止。
    | %#codegen
    | arg_arg_thrust=arg_arg_command;arg_arg_filter=arg_arg_oldFilter;
    | if arg_branch==3,arg_arg_filter=single(0);elseif arg_arg_manual,arg_arg_filter=arg_arg_command;end
    | if arg_arg_velEnable
    |  arg_arg_filter=filterStep(single(double(arg_arg_base+arg_arg_correction)*3.7),arg_arg_dt,single(.01),arg_arg_filter);arg_arg_thrust=arg_arg_filter;
    |  if arg_arg_auto && arg_arg_flipFlag==0
    |   if double(arg_arg_thrust)/3.7>double(single(arg_arg_base*single(1.15))),arg_arg_thrust=single(3.7*double(arg_arg_base)*double(single(1.15)));end
    |   if double(arg_arg_thrust)/3.7<double(single(arg_arg_base*single(.85))),arg_arg_thrust=single(3.7*double(arg_arg_base)*double(single(.85)));end
    |  end
    | end
    | if arg_branch==3,arg_arg_thrust=arg_arg_lastThrust;arg_arg_last=arg_arg_lastThrust;else,arg_arg_last=arg_arg_thrust;end
    | end
    | function s=filterStep(u,h,T,s),s=s*T/(T+h)+u*h/(T+h);end

== stateflow chart StampFly_StudentBlocks/LoggingAndStatus/StatusIndicators400 ==
  note: LED・ブザー：校正、待機、飛行、低電圧、通信異常とモード変更を表示。色・周波数・再起動判定はモデル内。ハードウェアブロックは受け取った値だけを出力。
  state Calculate
    en: [color1,color2,tone,restart]=stepFn(mode,controlMode,altFlag,flipFlag,lowVoltage,rcError,ahrsFlag,button);
    du: [color1,color2,tone,restart]=stepFn(mode,controlMode,altFlag,flipFlag,lowVoltage,rcError,ahrsFlag,button);
  (default) -> Calculate
  data: arg_mode function_input; arg_controlMode function_input; arg_altFlag function_input; arg_flipFlag function_input; arg_lowVoltage function_input; arg_rcError function_input; arg_ahrsFlag function_input; arg_button function_input; arg_color1 function_output; arg_color2 function_output; arg_tone function_output; arg_restart function_output; mode input uint8; controlMode input single; altFlag input uint8; flipFlag input uint8; lowVoltage input uint8; rcError input uint8; ahrsFlag input uint8; button input uint8; color1 output uint32; color2 output uint32; tone output uint32; restart output boolean
  function [arg_color1,arg_color2,arg_tone,arg_restart]=stepFn(arg_mode,arg_controlMode,arg_altFlag,arg_flipFlag,arg_lowVoltage,arg_rcError,arg_ahrsFlag,arg_button):
    | function [arg_color1,arg_color2,arg_tone,arg_restart]=stepFn(arg_mode,arg_controlMode,arg_altFlag,arg_flipFlag,arg_lowVoltage,arg_rcError,arg_ahrsFlag,arg_button)
    | % 公式led_driveの状態色。ブザーの200ms待機は400Hzカウンターへ置換。
    | %#codegen
    | persistent Blink Rainbow C1 C2 Tick AHRSPrev ToneTicks ButtonCount WasPressed;
    | if isempty(Blink)
    |  Blink=uint16(0);Rainbow=uint32(255);C1=uint32(0);C2=uint32(0);Tick=uint16(0);AHRSPrev=uint8(0);ToneTicks=uint16(0);ButtonCount=uint8(0);WasPressed=false;
    | end
    | if arg_mode==1,C1=uint32(hex2dec('FF00FF'));C2=C1;
    | elseif arg_mode==5,C1=uint32(hex2dec('00FF00'));C2=C1;
    | elseif arg_mode==2
    |  c=uint32(hex2dec('FFFF00'));
    |  if arg_controlMode~=0,c=uint32(hex2dec('DC669B'));elseif arg_flipFlag~=0,c=uint32(hex2dec('FF9933'));end
    |  if arg_altFlag>=1,c=uint32(hex2dec('331155'));end
    |  if arg_rcError==1,c=uint32(hex2dec('FF0000'));end
    |  C1=c;C2=c;if arg_lowVoltage>=100,C1=uint32(hex2dec('18EBF9'));end
    | elseif arg_mode==3
    |  if arg_lowVoltage<100
    |   if Blink==0
    |    top=bitand(Rainbow,uint32(hex2dec('800000')))~=0;Rainbow=bitshift(Rainbow,1);if top,Rainbow=bitor(Rainbow,uint32(1));end
    |    C1=Rainbow;C2=Rainbow;Blink=Blink+uint16(1);
    |   end
    |   Blink=Blink+uint16(1);if Blink>20,Blink=uint16(0);end
    |  else
    |   if Blink<10,C1=uint32(hex2dec('18EBF9'));C2=C1;
    |   elseif Blink<200,C1=uint32(0);C2=uint32(0);else,Blink=uint16(0);end
    |   Blink=Blink+uint16(1);
    |  end
    |  if arg_ahrsFlag~=AHRSPrev && arg_ahrsFlag==1,ToneTicks=uint16(80);end
    |  AHRSPrev=arg_ahrsFlag;
    | end
    | arg_tone=uint32(0);
    | % Startup notes from official buzzer.h. Four 200ms notes, then silence.
    | if Tick<320
    |  notes=uint32([294 441 350 393]);idx=min(floor(double(Tick)/80)+1,4);arg_tone=notes(idx);Tick=Tick+uint16(1);
    | elseif ToneTicks>0,arg_tone=uint32(4000);ToneTicks=ToneTicks-uint16(1);end
    | arg_restart=false;
    | if arg_button==1,ButtonCount=min(ButtonCount+uint8(1),uint8(40));if ButtonCount>=4,WasPressed=true;end
    | elseif WasPressed,arg_restart=true;WasPressed=false;ButtonCount=uint8(0);else,ButtonCount=uint8(0);end
    | % FastLED brightness15, show32: cap displayed channels without changing logic.
    | arg_color1=scale(C1);arg_color2=scale(C2);
    | end
    | function c=scale(x)
    | r=bitand(bitshift(x,-16),uint32(255));g=bitand(bitshift(x,-8),uint32(255));b=bitand(x,uint32(255));
    | c=bitor(bitor(bitshift(uint32(double(r)*15/255),16),bitshift(uint32(double(g)*15/255),8)),uint32(double(b)*15/255));
    | end

== stateflow chart StampFly_StudentBlocks/LoggingAndStatus/OfficialTelemetryValues ==
  note: 公式 JoyStick 用のテレメトリ：姿勢・角速度・PID診断・電圧・高度などを公式の順に整列。40 Hz ブロックがパケットを送信キューへ入れる。
  state Calculate
    en: [values]=stepFn(t,dt,a,r,cd,accel,voltage,duty,z,sd,v);
    du: [values]=stepFn(t,dt,a,r,cd,accel,voltage,duty,z,sd,v);
  (default) -> Calculate
  data: arg_t function_input; arg_dt function_input; arg_a function_input; arg_r function_input; arg_cd function_input; arg_accel function_input; arg_voltage function_input; arg_duty function_input; arg_z function_input; arg_sd function_input; arg_v function_input; arg_values function_output; t input single; dt input single; a input single; r input single; cd input single; accel input single; voltage input single; duty input single; z input single; sd input single; v input single; values output single
  function arg_values=stepFn(arg_t,arg_dt,arg_a,arg_r,arg_cd,arg_accel,arg_voltage,arg_duty,arg_z,arg_sd,arg_v):
    | function arg_values=stepFn(arg_t,arg_dt,arg_a,arg_r,arg_cd,arg_accel,arg_voltage,arg_duty,arg_z,arg_sd,arg_v)
    | % 公式120byteテレメトリの27個のfloat。バイト送信は専用IOブロック。
    | %#codegen
    | arg_values=zeros(27,1,'single');arg_values(1:2)=[arg_t;arg_dt];arg_values(3:8)=[arg_a;arg_r]*single(180/pi);
    | arg_values(9:13)=arg_cd(6:10)*single(180/pi);arg_values(14)=single(double(arg_cd(5))/3.7);
    | arg_values(15)=arg_voltage;arg_values(16:18)=arg_accel([2 1 3])/single(9.80665);arg_values(18)=-arg_values(18);
    | arg_values(19:20)=[arg_v;arg_cd(4)];arg_values(21:22)=arg_duty(2:3);
    | arg_values(23:27)=[arg_cd(1);arg_z;arg_sd(3);arg_sd(1:2)];
    | end

== stateflow chart StampFly_StudentBlocks/LoggingAndStatus/JoyStickTelemetry40/OfficialTelemetryValues ==
  note: 公式 JoyStick 用のテレメトリ：姿勢・角速度・PID診断・電圧・高度などを公式の順に整列。40 Hz ブロックがパケットを送信キューへ入れる。
  state Calculate
    en: [values]=stepFn(t,dt,a,r,cd,accel,voltage,duty,z,sd,v);
    du: [values]=stepFn(t,dt,a,r,cd,accel,voltage,duty,z,sd,v);
  (default) -> Calculate
  data: arg_t function_input; arg_dt function_input; arg_a function_input; arg_r function_input; arg_cd function_input; arg_accel function_input; arg_voltage function_input; arg_duty function_input; arg_z function_input; arg_sd function_input; arg_v function_input; arg_values function_output; t input single; dt input single; a input single; r input single; cd input single; accel input single; voltage input single; duty input single; z input single; sd input single; v input single; values output single
  function arg_values=stepFn(arg_t,arg_dt,arg_a,arg_r,arg_cd,arg_accel,arg_voltage,arg_duty,arg_z,arg_sd,arg_v):
    | function arg_values=stepFn(arg_t,arg_dt,arg_a,arg_r,arg_cd,arg_accel,arg_voltage,arg_duty,arg_z,arg_sd,arg_v)
    | % 公式120byteテレメトリの27個のfloat。バイト送信は専用IOブロック。
    | %#codegen
    | arg_values=zeros(27,1,'single');arg_values(1:2)=[arg_t;arg_dt];arg_values(3:8)=[arg_a;arg_r]*single(180/pi);
    | arg_values(9:13)=arg_cd(6:10)*single(180/pi);arg_values(14)=single(double(arg_cd(5))/3.7);
    | arg_values(15)=arg_voltage;arg_values(16:18)=arg_accel([2 1 3])/single(9.80665);arg_values(18)=-arg_values(18);
    | arg_values(19:20)=[arg_v;arg_cd(4)];arg_values(21:22)=arg_duty(2:3);
    | arg_values(23:27)=[arg_cd(1);arg_z;arg_sd(3);arg_sd(1:2)];
    | end
